simulink model "TSPMe_SeriesParallel"  (R2023a)
settings: Solver=daessc  StartTime=0.0  StopTime=15e4
libraries: fl_lib x34, nesl_utility x24, BatteryLibrary_lib x5
settings Model: Creator=widana_d  LastModifiedBy=widana_d
settings SolverCC: SolverResetMethod=Robust
settings DataIOCC: SaveState=on
settings DebuggingCC: UnconnectedInputMsg=warning  UnconnectedOutputMsg=warning  UnconnectedLineMsg=warning
settings ModelReferenceCC: EnableRefExpFcnMdlSchedulingChecks=on
settings RTWCC: DLArmComputeVersion=19.05

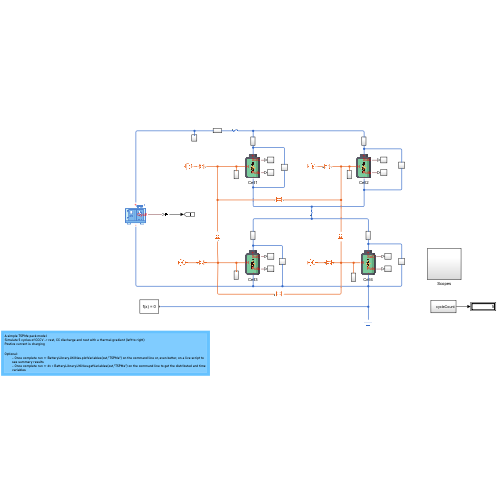
[thumbnail: Simulink's stored preview of the top-level diagram]
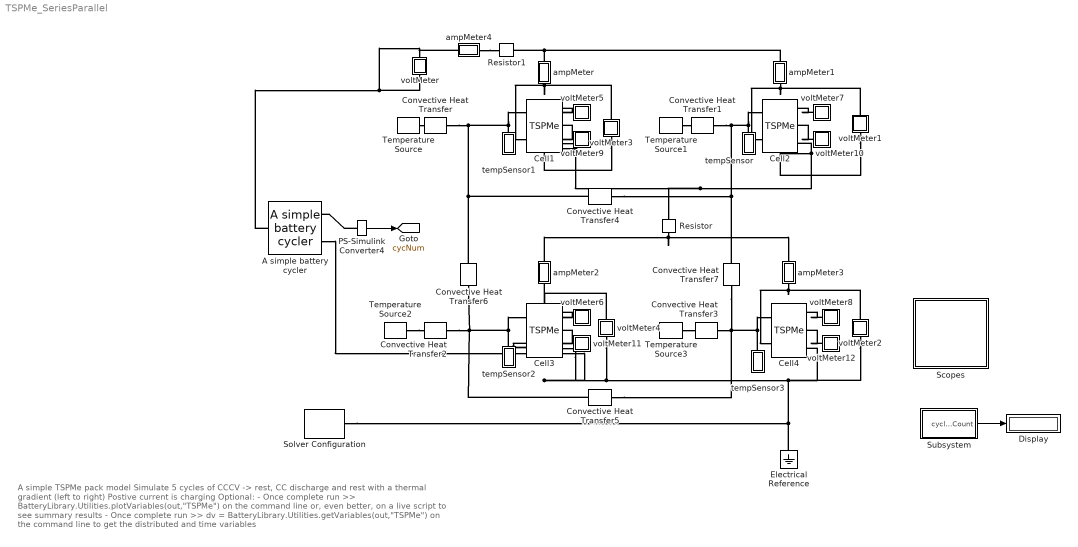
== system TSPMe_SeriesParallel ==
  note: A simple TSPMe pack model
      | Simulate 5 cycles of CCCV -> rest, CC discharge and rest with a thermal gradient (left to right)
      | Postive current is charging
      |
      | Optional:
      | - Once complete run >> BatteryLibrary.Utilities.plotVariables(out,"TSPMe") on the command line or, even better, on a live script to see summary results
      | - Once complete run >> dv = BatteryLibrary.Utilities.getVariables(out,"TSPMe") on the command line to get the distributed and time variables
  A simple battery cycler : BatteryLibrary_lib/Utilities/A simple battery cycler  Vmax=8.3 V  Vmin=5 V  Ic=4 A  Ico=0.5 A  Id=-10 A  tRestC=1800 s  tRestD=3600 s
      settings: InternalSimscapePortConfiguration="{\"Bottom\":[{\"id\":\"n\",\"label\":\"-\",\"type\":\"foundation.electrical.electrical\"}],\"Left\":[],\"Right\":[{\"id\":\"numCyc\",\"label\":\"Cyc#\",\"type\":\"output\"}],\"Top\":[{\"id\":\"p\",\"label\":\"+\",\"type\":\"foundation.electrical.electrical\"}]}"
  Cell{1..4} (4 alike) : BatteryLibrary_lib/Models/TSPMe  z0=0.4  T0=298 K  Cn=4.9 hr*A  DnRef=3.3E-14 m^2/s  DpRef=4E-15 m^2/s  sigma_eRef=1.2 S/m  tr=0.2594  ce0=1000 mol/m^3  cn_max=33133 mol/m^3  cp_max=63104 mol/m^3  sn_max=0.9014  sn_min=0.0279  sp_max=0.9072  sp_min=0.2567  knRef=6.48E-7 m^2.50000*A/mol^1.50000  kpRef=3.42E-6 m^2.50000*A/mol^1.50000  Cp=110 J/K  Tref=298 K  Ea_kn=1 kJ/mol  Ea_kp=1 kJ/mol  Ea_Dn=75 kJ/mol  Ea_Dp=10 kJ/mol  Ea_De=1.2 kJ/mol  Ea_sigmae=80 kJ/mol  Ln=85.2 um  Ls=12 um  Lp=75.6 um  Area_p=1027 cm^2  eps_n=0.25  eps_s=0.47  eps_p=0.335  Rn=5.86 um  Rp=5.22 um  an=3.84E5 1/m  ap=3.82E5 1/m
      settings: InternalSimscapePortConfiguration="{\"Bottom\":[{\"id\":\"n\",\"label\":\"-\",\"type\":\"foundation.electrical.electrical\"}],\"Left\":[{\"id\":\"Hi\",\"label\":\"H\",\"type\":\"foundation.thermal.thermal\"}],\"Right\":[{\"id\":\"z\",\"label\":\"SoC\",\"type\":\"output\"},{\"id\":\"pots\",\"label\":\"Pots\",\"type\":\"output\"}],\"Top\":[{\"id\":\"p\",\"label\":\"+\",\"type\":\"foundation.electrical.electrical\"}]}"
  Convective Heat Transfer{,1..3} (4 alike) : fl_lib/Thermal/Thermal Elements/Convective Heat Transfer  thermal_type=foundation.enum.constant_variable.constant  area=0.0023 m^2  heat_tr_coeff=35 W/(m^2 * K)  min_heat_tr_coeff=1e-3 W/(K*m^2)  T_specify=off  T_priority=None  T=0 K  T_nominal_specify=off  T_nominal_unit=K  T_nominal_value=1  Q_specify=off  Q_priority=None  Q=0 W  Q_nominal_specify=off  Q_nominal_unit=W  Q_nominal_value=1
  Convective Heat Transfer4 : fl_lib/Thermal/Thermal Elements/Convective Heat Transfer  thermal_type=foundation.enum.constant_variable.constant  area=0.0015 m^2  heat_tr_coeff=10 W/(m^2 * K)  min_heat_tr_coeff=1e-3 W/(K*m^2)  T_specify=off  T_priority=None  T=0 K  T_nominal_specify=off  T_nominal_unit=K  T_nominal_value=1  Q_specify=off  Q_priority=None  Q=0 W  Q_nominal_specify=off  Q_nominal_unit=W  Q_nominal_value=1
  Convective Heat Transfer5 : fl_lib/Thermal/Thermal Elements/Convective Heat Transfer  thermal_type=foundation.enum.constant_variable.constant  area=0.00115 m^2  heat_tr_coeff=10 W/(m^2 * K)  min_heat_tr_coeff=1e-3 W/(K*m^2)  T_specify=off  T_priority=None  T=0 K  T_nominal_specify=off  T_nominal_unit=K  T_nominal_value=1  Q_specify=off  Q_priority=None  Q=0 W  Q_nominal_specify=off  Q_nominal_unit=W  Q_nominal_value=1
  Convective Heat Transfer6 : fl_lib/Thermal/Thermal Elements/Convective Heat Transfer  thermal_type=foundation.enum.constant_variable.constant  area=0.00115 m^2  heat_tr_coeff=10 W/(m^2 * K)  min_heat_tr_coeff=1e-3 W/(K*m^2)  T_specify=off  T_priority=None  T=0 K  T_nominal_specify=off  T_nominal_unit=K  T_nominal_value=1  Q_specify=off  Q_priority=None  Q=0 W  Q_nominal_specify=off  Q_nominal_unit=W  Q_nominal_value=1
  Convective Heat Transfer7 : fl_lib/Thermal/Thermal Elements/Convective Heat Transfer  thermal_type=foundation.enum.constant_variable.constant  area=0.00115 m^2  heat_tr_coeff=10 W/(m^2 * K)  min_heat_tr_coeff=1e-3 W/(K*m^2)  T_specify=off  T_priority=None  T=0 K  T_nominal_specify=off  T_nominal_unit=K  T_nominal_value=1  Q_specify=off  Q_priority=None  Q=0 W  Q_nominal_specify=off  Q_nominal_unit=W  Q_nominal_value=1
  Display : Display
  Electrical Reference : fl_lib/Electrical/Electrical Elements/Electrical Reference
  PS-Simulink Converter4 : nesl_utility/PS-Simulink Converter  PhysicalDomain=network_engine_domain  SubClassName=ps_output  LeftPortType=input  RightPortType=output  PseudoPeriodic=off  Frequencies=[]  VectorFormat=1-D array  Unit=inherit  AffineConversion=off
  Resistor : fl_lib/Electrical/Electrical Elements/Resistor  R=1e-3 Ohm  i_specify=off  i_priority=None  i=0 A  i_nominal_specify=off  i_nominal_unit=A  i_nominal_value=1  v_specify=off  v_priority=None  v=0 V  v_nominal_specify=off  v_nominal_unit=V  v_nominal_value=1
  Resistor1 : fl_lib/Electrical/Electrical Elements/Resistor  R=1e-3 Ohm  i_specify=off  i_priority=None  i=0 A  i_nominal_specify=off  i_nominal_unit=A  i_nominal_value=1  v_specify=off  v_priority=None  v=0 V  v_nominal_specify=off  v_nominal_unit=V  v_nominal_value=1
  Scopes : Subsystem
  Solver Configuration : nesl_utility/Solver Configuration  PhysicalDomain=network_engine_domain  SubClassName=solver  LeftPortType=input  RightPortType=generic  Tones=[]  Harmonics=[]  SimulateNoise=off  Profile=off  UseLocalSampling=off  EnableSwitchedLinearOptims=on  FrequencyDomain=off  UseCCode=off  RelTol=0.001  AbsTol=1e-06  MinStep=1e-09  ToWorkspace=off  RevertToSquareIcSolve=off  NumHomotopyIterations=100  PhasorMode=off  PhasorModeNumHarmonics=1  ConsistencySolver=NEWTON_FTOL  IndexReductionMethod=DerivativeReplacement  DoDC=off  ResidualTolerance=1e-09  ConsistencyTolSource=GLOBAL  ConsistencyAbsTol=0.001  ConsistencyRelTol=0.001  ConsistencyTolFactor=0.001  UseLocalSolver=off  LocalSolverChoice=NE_BACKWARD_EULER_ADVANCER  ResolveIndetEquations=on  FunctionEvalNumThread=1  LocalSolverSampleTime=0.001  DoFixedCost=off  MaxNonlinIter=3  MaxModeIter=2  ComputeImpulses=off  ImpulseIterations=2  LinearAlgebra=auto  LinearAlgebraNumThread=0  EquationFormulation=NE_TIME_EF  DelaysMemoryBudget=1024  AutomaticFiltering=on  FilteringTimeConstant=0.001  PartitionStorageMethod=AS_NEEDED  PartitionMemoryBudget=1024  PartitionMethod=ROBUST
  Subsystem : Subsystem
  Temperature Source : fl_lib/Thermal/Thermal Sources/Temperature Source  temperature=30 degC
  Temperature Source1 : fl_lib/Thermal/Thermal Sources/Temperature Source  temperature=20 degC
  Temperature Source2 : fl_lib/Thermal/Thermal Sources/Temperature Source  temperature=30 degC
  Temperature Source3 : fl_lib/Thermal/Thermal Sources/Temperature Source  temperature=20 degC
  ampMeter : Subsystem
  ampMeter1 : Subsystem
  ampMeter2 : Subsystem
  ampMeter3 : Subsystem
  ampMeter4 : Subsystem
  tempSensor : Subsystem
  tempSensor1 : Subsystem
  tempSensor2 : Subsystem
  tempSensor3 : Subsystem
  voltMeter : Subsystem
  voltMeter1 : Subsystem
  voltMeter10 : Subsystem
  voltMeter11 : Subsystem
  voltMeter12 : Subsystem
  voltMeter2 : Subsystem
  voltMeter3 : Subsystem
  voltMeter4 : Subsystem
  voltMeter5 : Subsystem
  voltMeter6 : Subsystem
  voltMeter7 : Subsystem
  voltMeter8 : Subsystem
  voltMeter9 : Subsystem
  tag scope: cycNum=global
  wires:
  Subsystem/1(cycleCount) -> Display/1
  PS-Simulink Converter4/1 -> [cycNum]
  connections:
  Temperature Source/LConn1 -- Convective Heat Transfer/RConn1
  A simple battery cycler/LConn1 -- voltMeter/LConn1 -- ampMeter4/LConn1
  Temperature Source2/LConn1 -- Convective Heat Transfer2/RConn1
  PS-Simulink Converter4/LConn1 -- A simple battery cycler/RConn1
  ampMeter4/RConn1 -- Resistor1/LConn1
  tempSensor1/LConn1 -- Convective Heat Transfer6/LConn1 -- Convective Heat Transfer4/RConn1 -- Convective Heat Transfer/LConn1 -- Cell1/LConn1
  ampMeter/LConn1 -- Resistor1/RConn1 -- ampMeter1/LConn1
  Convective Heat Transfer2/LConn1 -- Convective Heat Transfer6/RConn1 -- tempSensor2/LConn1 -- Cell3/LConn1 -- Convective Heat Transfer5/RConn1
  voltMeter11/LConn1 -- Cell3/RConn2
  Cell1/RConn3 -- voltMeter3/RConn1 -- Resistor/RConn1 -- voltMeter1/RConn1 -- Cell2/RConn3
  voltMeter6/LConn1 -- Cell3/RConn1
  voltMeter10/LConn1 -- Cell2/RConn2
  ampMeter2/LConn1 -- Resistor/LConn1 -- ampMeter3/LConn1
  ampMeter3/RConn1 -- voltMeter2/LConn1 -- Cell4/LConn2
  Temperature Source3/LConn1 -- Convective Heat Transfer3/RConn1
  ampMeter/RConn1 -- voltMeter3/LConn1 -- Cell1/LConn2
  Temperature Source1/LConn1 -- Convective Heat Transfer1/RConn1
  voltMeter12/LConn1 -- Cell4/RConn2
  ampMeter1/RConn1 -- voltMeter1/LConn1 -- Cell2/LConn2
  voltMeter4/RConn1 -- Cell3/RConn3 -- A simple battery cycler/RConn2 -- Cell4/RConn3 -- Solver Configuration/RConn1 -- Electrical Reference/LConn1 -- voltMeter2/RConn1
  voltMeter8/LConn1 -- Cell4/RConn1
  Convective Heat Transfer3/LConn1 -- Cell4/LConn1 -- tempSensor3/LConn1 -- Convective Heat Transfer5/LConn1 -- Convective Heat Transfer7/RConn1
  voltMeter7/LConn1 -- Cell2/RConn1
  Convective Heat Transfer1/LConn1 -- Convective Heat Transfer4/LConn1 -- Convective Heat Transfer7/LConn1 -- tempSensor/LConn1 -- Cell2/LConn1
  voltMeter5/LConn1 -- Cell1/RConn1
  Cell3/LConn2 -- voltMeter4/LConn1 -- ampMeter2/RConn1
  voltMeter9/LConn1 -- Cell1/RConn2

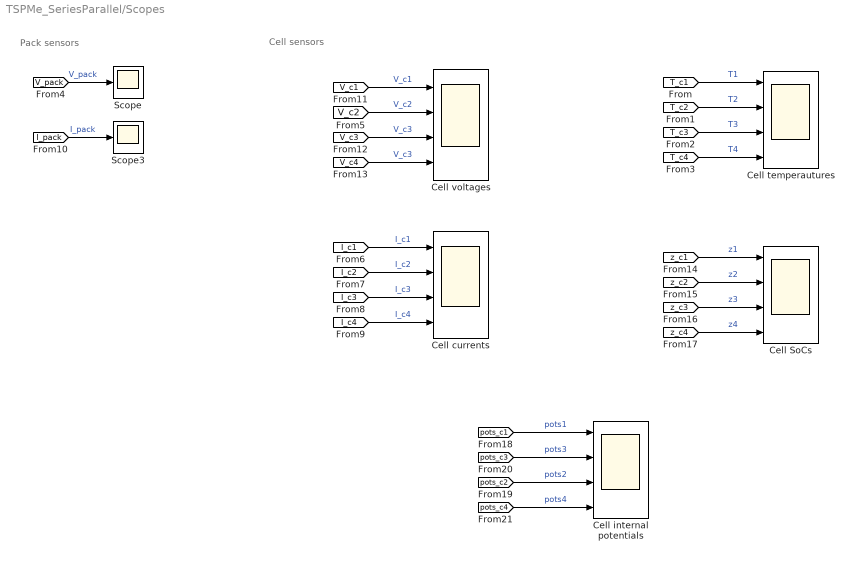
== system TSPMe_SeriesParallel/Scopes ==
  note: Cell sensors
  note: Pack sensors
  Cell SoCs : Scope  NumInputPorts=4
  Cell currents : Scope  NumInputPorts=4
  Cell internal potentials : Scope  NumInputPorts=4
  Cell temperautures : Scope  NumInputPorts=4
  Cell voltages : Scope  NumInputPorts=4
  Scope : Scope
  Scope3 : Scope
  wires:
  [I_c2] -> Cell currents/2  "I_c2"
  [V_c1] -> Cell voltages/1  "V_c1"
  [I_pack] -> Scope3/1  "I_pack"
  [I_c3] -> Cell currents/3  "I_c3"
  [V_c2] -> Cell voltages/2  "V_c2"
  [V_c4] -> Cell voltages/4  "V_c3"
  [V_pack] -> Scope/1  "V_pack"
  [V_c3] -> Cell voltages/3  "V_c3"
  [I_c4] -> Cell currents/4  "I_c4"
  [I_c1] -> Cell currents/1  "I_c1"
  [T_c2] -> Cell temperautures/2  "T2"
  [T_c1] -> Cell temperautures/1  "T1"
  [T_c3] -> Cell temperautures/3  "T3"
  [T_c4] -> Cell temperautures/4  "T4"
  [z_c3] -> Cell SoCs/3  "z3"
  [z_c4] -> Cell SoCs/4  "z4"
  [z_c1] -> Cell SoCs/1  "z1"
  [z_c2] -> Cell SoCs/2  "z2"
  [pots_c2] -> Cell internal potentials/3  "pots2"
  [pots_c1] -> Cell internal potentials/1  "pots1"
  [pots_c4] -> Cell internal potentials/4  "pots4"
  [pots_c3] -> Cell internal potentials/2  "pots3"

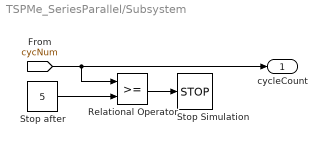
== system TSPMe_SeriesParallel/Subsystem ==
  Relational Operator : RelationalOperator  OutDataTypeStr=boolean  RndMeth=Simplest  InputSameDT=off
  Stop Simulation : Stop
  Stop after : Constant  Value=5
  cycleCount : Outport
  wires:
  Stop after/1 -> Relational Operator/2
  [cycNum] -> cycleCount/1, Relational Operator/1
  Relational Operator/1 -> Stop Simulation/1

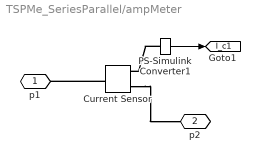
== system TSPMe_SeriesParallel/ampMeter ==
  Current Sensor : fl_lib/Electrical/Electrical Sensors/Current Sensor
  PS-Simulink Converter1 : nesl_utility/PS-Simulink Converter  PhysicalDomain=network_engine_domain  SubClassName=ps_output  LeftPortType=input  RightPortType=output  PseudoPeriodic=off  Frequencies=[]  VectorFormat=1-D array  Unit=inherit  AffineConversion=off
  p1 : PMIOPort  Side=Left
  p2 : PMIOPort  Port=2  Side=Right
  tag scope: I_c1=global
  wires:
  PS-Simulink Converter1/1 -> [I_c1]
  connections:
  Current Sensor/RConn2 -- p2/RConn1
  Current Sensor/LConn1 -- p1/RConn1
  PS-Simulink Converter1/LConn1 -- Current Sensor/RConn1

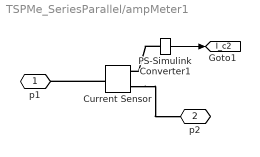
== system TSPMe_SeriesParallel/ampMeter1 ==
  Current Sensor : fl_lib/Electrical/Electrical Sensors/Current Sensor
  PS-Simulink Converter1 : nesl_utility/PS-Simulink Converter  PhysicalDomain=network_engine_domain  SubClassName=ps_output  LeftPortType=input  RightPortType=output  PseudoPeriodic=off  Frequencies=[]  VectorFormat=1-D array  Unit=inherit  AffineConversion=off
  p1 : PMIOPort  Side=Left
  p2 : PMIOPort  Port=2  Side=Right
  tag scope: I_c2=global
  wires:
  PS-Simulink Converter1/1 -> [I_c2]
  connections:
  Current Sensor/RConn2 -- p2/RConn1
  Current Sensor/LConn1 -- p1/RConn1
  PS-Simulink Converter1/LConn1 -- Current Sensor/RConn1

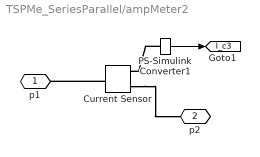
== system TSPMe_SeriesParallel/ampMeter2 ==
  Current Sensor : fl_lib/Electrical/Electrical Sensors/Current Sensor
  PS-Simulink Converter1 : nesl_utility/PS-Simulink Converter  PhysicalDomain=network_engine_domain  SubClassName=ps_output  LeftPortType=input  RightPortType=output  PseudoPeriodic=off  Frequencies=[]  VectorFormat=1-D array  Unit=inherit  AffineConversion=off
  p1 : PMIOPort  Side=Left
  p2 : PMIOPort  Port=2  Side=Right
  tag scope: I_c3=global
  wires:
  PS-Simulink Converter1/1 -> [I_c3]
  connections:
  Current Sensor/RConn2 -- p2/RConn1
  Current Sensor/LConn1 -- p1/RConn1
  PS-Simulink Converter1/LConn1 -- Current Sensor/RConn1

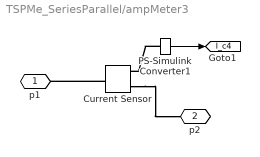
== system TSPMe_SeriesParallel/ampMeter3 ==
  Current Sensor : fl_lib/Electrical/Electrical Sensors/Current Sensor
  PS-Simulink Converter1 : nesl_utility/PS-Simulink Converter  PhysicalDomain=network_engine_domain  SubClassName=ps_output  LeftPortType=input  RightPortType=output  PseudoPeriodic=off  Frequencies=[]  VectorFormat=1-D array  Unit=inherit  AffineConversion=off
  p1 : PMIOPort  Side=Left
  p2 : PMIOPort  Port=2  Side=Right
  tag scope: I_c4=global
  wires:
  PS-Simulink Converter1/1 -> [I_c4]
  connections:
  Current Sensor/RConn2 -- p2/RConn1
  Current Sensor/LConn1 -- p1/RConn1
  PS-Simulink Converter1/LConn1 -- Current Sensor/RConn1

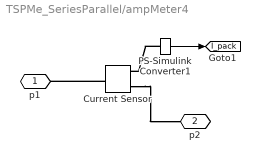
== system TSPMe_SeriesParallel/ampMeter4 ==
  Current Sensor : fl_lib/Electrical/Electrical Sensors/Current Sensor
  PS-Simulink Converter1 : nesl_utility/PS-Simulink Converter  PhysicalDomain=network_engine_domain  SubClassName=ps_output  LeftPortType=input  RightPortType=output  PseudoPeriodic=off  Frequencies=[]  VectorFormat=1-D array  Unit=inherit  AffineConversion=off
  p1 : PMIOPort  Side=Left
  p2 : PMIOPort  Port=2  Side=Right
  tag scope: I_pack=global
  wires:
  PS-Simulink Converter1/1 -> [I_pack]
  connections:
  Current Sensor/RConn2 -- p2/RConn1
  Current Sensor/LConn1 -- p1/RConn1
  PS-Simulink Converter1/LConn1 -- Current Sensor/RConn1

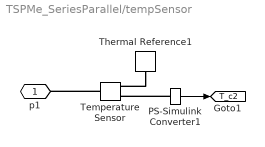
== system TSPMe_SeriesParallel/tempSensor ==
  PS-Simulink Converter1 : nesl_utility/PS-Simulink Converter  PhysicalDomain=network_engine_domain  SubClassName=ps_output  LeftPortType=input  RightPortType=output  PseudoPeriodic=off  Frequencies=[]  VectorFormat=1-D array  Unit=inherit  AffineConversion=off
  Temperature Sensor : fl_lib/Thermal/Thermal Sensors/Temperature Sensor  temperature_measure=foundation.enum.MeasurementReference.difference
  Thermal Reference1 : fl_lib/Thermal/Thermal Elements/Thermal Reference
  p1 : PMIOPort  Side=Left
  tag scope: T_c2=global
  wires:
  PS-Simulink Converter1/1 -> [T_c2]
  connections:
  Temperature Sensor/LConn1 -- p1/RConn1
  PS-Simulink Converter1/LConn1 -- Temperature Sensor/RConn2
  Thermal Reference1/LConn1 -- Temperature Sensor/RConn1

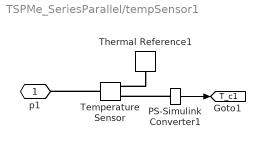
== system TSPMe_SeriesParallel/tempSensor1 ==
  PS-Simulink Converter1 : nesl_utility/PS-Simulink Converter  PhysicalDomain=network_engine_domain  SubClassName=ps_output  LeftPortType=input  RightPortType=output  PseudoPeriodic=off  Frequencies=[]  VectorFormat=1-D array  Unit=inherit  AffineConversion=off
  Temperature Sensor : fl_lib/Thermal/Thermal Sensors/Temperature Sensor  temperature_measure=foundation.enum.MeasurementReference.difference
  Thermal Reference1 : fl_lib/Thermal/Thermal Elements/Thermal Reference
  p1 : PMIOPort  Side=Left
  tag scope: T_c1=global
  wires:
  PS-Simulink Converter1/1 -> [T_c1]
  connections:
  Temperature Sensor/LConn1 -- p1/RConn1
  PS-Simulink Converter1/LConn1 -- Temperature Sensor/RConn2
  Thermal Reference1/LConn1 -- Temperature Sensor/RConn1

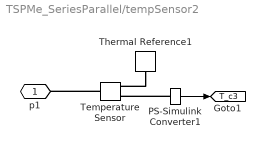
== system TSPMe_SeriesParallel/tempSensor2 ==
  PS-Simulink Converter1 : nesl_utility/PS-Simulink Converter  PhysicalDomain=network_engine_domain  SubClassName=ps_output  LeftPortType=input  RightPortType=output  PseudoPeriodic=off  Frequencies=[]  VectorFormat=1-D array  Unit=inherit  AffineConversion=off
  Temperature Sensor : fl_lib/Thermal/Thermal Sensors/Temperature Sensor  temperature_measure=foundation.enum.MeasurementReference.difference
  Thermal Reference1 : fl_lib/Thermal/Thermal Elements/Thermal Reference
  p1 : PMIOPort  Side=Left
  tag scope: T_c3=global
  wires:
  PS-Simulink Converter1/1 -> [T_c3]
  connections:
  Temperature Sensor/LConn1 -- p1/RConn1
  PS-Simulink Converter1/LConn1 -- Temperature Sensor/RConn2
  Thermal Reference1/LConn1 -- Temperature Sensor/RConn1

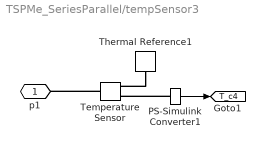
== system TSPMe_SeriesParallel/tempSensor3 ==
  PS-Simulink Converter1 : nesl_utility/PS-Simulink Converter  PhysicalDomain=network_engine_domain  SubClassName=ps_output  LeftPortType=input  RightPortType=output  PseudoPeriodic=off  Frequencies=[]  VectorFormat=1-D array  Unit=inherit  AffineConversion=off
  Temperature Sensor : fl_lib/Thermal/Thermal Sensors/Temperature Sensor  temperature_measure=foundation.enum.MeasurementReference.difference
  Thermal Reference1 : fl_lib/Thermal/Thermal Elements/Thermal Reference
  p1 : PMIOPort  Side=Left
  tag scope: T_c4=global
  wires:
  PS-Simulink Converter1/1 -> [T_c4]
  connections:
  Temperature Sensor/LConn1 -- p1/RConn1
  PS-Simulink Converter1/LConn1 -- Temperature Sensor/RConn2
  Thermal Reference1/LConn1 -- Temperature Sensor/RConn1

== system TSPMe_SeriesParallel/voltMeter ==
  Electrical Reference1 : fl_lib/Electrical/Electrical Elements/Electrical Reference
  PS-Simulink Converter : nesl_utility/PS-Simulink Converter  PhysicalDomain=network_engine_domain  SubClassName=ps_output  LeftPortType=input  RightPortType=output  PseudoPeriodic=off  Frequencies=[]  VectorFormat=1-D array  Unit=inherit  AffineConversion=off
  Voltage Sensor : fl_lib/Electrical/Electrical Sensors/Voltage Sensor
  Conn1 : PMIOPort  Side=Left
  tag scope: V_pack=global
  wires:
  PS-Simulink Converter/1 -> [V_pack]  "V"
  connections:
  Voltage Sensor/LConn1 -- Conn1/RConn1
  PS-Simulink Converter/LConn1 -- Voltage Sensor/RConn1
  Electrical Reference1/LConn1 -- Voltage Sensor/RConn2

== system TSPMe_SeriesParallel/voltMeter1 ==
  PS-Simulink Converter : nesl_utility/PS-Simulink Converter  PhysicalDomain=network_engine_domain  SubClassName=ps_output  LeftPortType=input  RightPortType=output  PseudoPeriodic=off  Frequencies=[]  VectorFormat=1-D array  Unit=inherit  AffineConversion=off
  Voltage Sensor : fl_lib/Electrical/Electrical Sensors/Voltage Sensor
  p1 : PMIOPort  Side=Left
  p2 : PMIOPort  Port=2  Side=Right
  tag scope: V_c2=global
  wires:
  PS-Simulink Converter/1 -> [V_c2]  "V"
  connections:
  Voltage Sensor/LConn1 -- p1/RConn1
  PS-Simulink Converter/LConn1 -- Voltage Sensor/RConn1
  p2/RConn1 -- Voltage Sensor/RConn2

== system TSPMe_SeriesParallel/voltMeter10 ==
  PS-Simulink Converter : nesl_utility/PS-Simulink Converter  PhysicalDomain=network_engine_domain  SubClassName=ps_output  LeftPortType=input  RightPortType=output  PseudoPeriodic=off  Frequencies=[]  VectorFormat=1-D array  Unit=inherit  AffineConversion=off
  p1 : PMIOPort  Side=Left
  tag scope: pots_c2=global
  wires:
  PS-Simulink Converter/1 -> [pots_c2]  "V"
  connections:
  p1/RConn1 -- PS-Simulink Converter/LConn1

== system TSPMe_SeriesParallel/voltMeter11 ==
  PS-Simulink Converter : nesl_utility/PS-Simulink Converter  PhysicalDomain=network_engine_domain  SubClassName=ps_output  LeftPortType=input  RightPortType=output  PseudoPeriodic=off  Frequencies=[]  VectorFormat=1-D array  Unit=inherit  AffineConversion=off
  p1 : PMIOPort  Side=Left
  tag scope: pots_c3=global
  wires:
  PS-Simulink Converter/1 -> [pots_c3]  "V"
  connections:
  p1/RConn1 -- PS-Simulink Converter/LConn1

== system TSPMe_SeriesParallel/voltMeter12 ==
  PS-Simulink Converter : nesl_utility/PS-Simulink Converter  PhysicalDomain=network_engine_domain  SubClassName=ps_output  LeftPortType=input  RightPortType=output  PseudoPeriodic=off  Frequencies=[]  VectorFormat=1-D array  Unit=inherit  AffineConversion=off
  p1 : PMIOPort  Side=Left
  tag scope: pots_c4=global
  wires:
  PS-Simulink Converter/1 -> [pots_c4]  "V"
  connections:
  p1/RConn1 -- PS-Simulink Converter/LConn1

== system TSPMe_SeriesParallel/voltMeter2 ==
  PS-Simulink Converter : nesl_utility/PS-Simulink Converter  PhysicalDomain=network_engine_domain  SubClassName=ps_output  LeftPortType=input  RightPortType=output  PseudoPeriodic=off  Frequencies=[]  VectorFormat=1-D array  Unit=inherit  AffineConversion=off
  Voltage Sensor : fl_lib/Electrical/Electrical Sensors/Voltage Sensor
  p1 : PMIOPort  Side=Left
  p2 : PMIOPort  Port=2  Side=Right
  tag scope: V_c4=global
  wires:
  PS-Simulink Converter/1 -> [V_c4]  "V"
  connections:
  Voltage Sensor/LConn1 -- p1/RConn1
  PS-Simulink Converter/LConn1 -- Voltage Sensor/RConn1
  p2/RConn1 -- Voltage Sensor/RConn2

== system TSPMe_SeriesParallel/voltMeter3 ==
  PS-Simulink Converter : nesl_utility/PS-Simulink Converter  PhysicalDomain=network_engine_domain  SubClassName=ps_output  LeftPortType=input  RightPortType=output  PseudoPeriodic=off  Frequencies=[]  VectorFormat=1-D array  Unit=inherit  AffineConversion=off
  Voltage Sensor : fl_lib/Electrical/Electrical Sensors/Voltage Sensor
  p1 : PMIOPort  Side=Left
  p2 : PMIOPort  Port=2  Side=Right
  tag scope: V_c1=global
  wires:
  PS-Simulink Converter/1 -> [V_c1]  "V"
  connections:
  Voltage Sensor/LConn1 -- p1/RConn1
  PS-Simulink Converter/LConn1 -- Voltage Sensor/RConn1
  p2/RConn1 -- Voltage Sensor/RConn2

== system TSPMe_SeriesParallel/voltMeter4 ==
  PS-Simulink Converter : nesl_utility/PS-Simulink Converter  PhysicalDomain=network_engine_domain  SubClassName=ps_output  LeftPortType=input  RightPortType=output  PseudoPeriodic=off  Frequencies=[]  VectorFormat=1-D array  Unit=inherit  AffineConversion=off
  Voltage Sensor : fl_lib/Electrical/Electrical Sensors/Voltage Sensor
  p1 : PMIOPort  Side=Left
  p2 : PMIOPort  Port=2  Side=Right
  tag scope: V_c3=global
  wires:
  PS-Simulink Converter/1 -> [V_c3]  "V"
  connections:
  Voltage Sensor/LConn1 -- p1/RConn1
  PS-Simulink Converter/LConn1 -- Voltage Sensor/RConn1
  p2/RConn1 -- Voltage Sensor/RConn2

== system TSPMe_SeriesParallel/voltMeter5 ==
  PS-Simulink Converter : nesl_utility/PS-Simulink Converter  PhysicalDomain=network_engine_domain  SubClassName=ps_output  LeftPortType=input  RightPortType=output  PseudoPeriodic=off  Frequencies=[]  VectorFormat=1-D array  Unit=inherit  AffineConversion=off
  p1 : PMIOPort  Side=Left
  tag scope: z_c1=global
  wires:
  PS-Simulink Converter/1 -> [z_c1]  "V"
  connections:
  p1/RConn1 -- PS-Simulink Converter/LConn1

== system TSPMe_SeriesParallel/voltMeter6 ==
  PS-Simulink Converter : nesl_utility/PS-Simulink Converter  PhysicalDomain=network_engine_domain  SubClassName=ps_output  LeftPortType=input  RightPortType=output  PseudoPeriodic=off  Frequencies=[]  VectorFormat=1-D array  Unit=inherit  AffineConversion=off
  p1 : PMIOPort  Side=Left
  tag scope: z_c3=global
  wires:
  PS-Simulink Converter/1 -> [z_c3]  "V"
  connections:
  p1/RConn1 -- PS-Simulink Converter/LConn1

== system TSPMe_SeriesParallel/voltMeter7 ==
  PS-Simulink Converter : nesl_utility/PS-Simulink Converter  PhysicalDomain=network_engine_domain  SubClassName=ps_output  LeftPortType=input  RightPortType=output  PseudoPeriodic=off  Frequencies=[]  VectorFormat=1-D array  Unit=inherit  AffineConversion=off
  p1 : PMIOPort  Side=Left
  tag scope: z_c2=global
  wires:
  PS-Simulink Converter/1 -> [z_c2]  "V"
  connections:
  p1/RConn1 -- PS-Simulink Converter/LConn1

== system TSPMe_SeriesParallel/voltMeter8 ==
  PS-Simulink Converter : nesl_utility/PS-Simulink Converter  PhysicalDomain=network_engine_domain  SubClassName=ps_output  LeftPortType=input  RightPortType=output  PseudoPeriodic=off  Frequencies=[]  VectorFormat=1-D array  Unit=inherit  AffineConversion=off
  p1 : PMIOPort  Side=Left
  tag scope: z_c4=global
  wires:
  PS-Simulink Converter/1 -> [z_c4]  "V"
  connections:
  p1/RConn1 -- PS-Simulink Converter/LConn1

== system TSPMe_SeriesParallel/voltMeter9 ==
  PS-Simulink Converter : nesl_utility/PS-Simulink Converter  PhysicalDomain=network_engine_domain  SubClassName=ps_output  LeftPortType=input  RightPortType=output  PseudoPeriodic=off  Frequencies=[]  VectorFormat=1-D array  Unit=inherit  AffineConversion=off
  p1 : PMIOPort  Side=Left
  tag scope: pots_c1=global
  wires:
  PS-Simulink Converter/1 -> [pots_c1]  "V"
  connections:
  p1/RConn1 -- PS-Simulink Converter/LConn1
